simulink model "top_integrated_nanogrid"  (R2026a)
settings: Solver=ode23t  StopTime=1
values from neighbouring files (symbols this model uses):
  irradiance_day = pchip(t_coarse, irradiance_coarse, t_sim)    [flc_init.m]
  t_sim = linspace(0, 1.0, 1001)    [flc_init.m]
undefined symbols (not defined in the file or in its folder): DiscIntNeverNeededParam
libraries: fl_lib x19, nesl_utility x14, ee_lib x13, slpidlib x2, batteryecm_lib x1, fuzblock x1, eePwmGenerator x1
(part 2 of 2)

== matlab function top_integrated_nanogrid/MPPT/MATLAB Function ==
  data: u input; y output
function y = scale_signal(u)
    % Scale [-60, 100] to [-1, 1] with input clamping
    u_clamped = min(max(u, -60), 100); 
    y = (u_clamped - 20) / 80;
end

== matlab function top_integrated_nanogrid/MANAGEMENT_SYSTEM/MATLAB Function ==
  data: P_solar input; Mode output; P_load input; SoC input; P_net output; Battery_Cmd output; Load_Status output
function [Mode, P_net, Battery_Cmd, Load_Status] = nanogrid_controller(P_solar, P_load, SoC)
% #codegen

% --- 1. DEFAULT INITIALIZATIONS (Prevents Undefined Output Errors) ---
Mode        = 1;     % Default to Mode 1
P_net       = 0;     % Default power balance
Battery_Cmd = 0;     % Default Battery Idle (0)
Load_Status = 1;     % Default Load Connected (1)

% --- 2. POWER CALCULATION ---
P_net = P_solar - P_load;

% --- 3. ENERGY MANAGEMENT LOGIC ---
if P_solar >= P_load
    % --- PV Generation Covers or Exceeds Demand ---
    if P_solar == P_load
        % MODE 1: Solar matches load demand perfectly
        Mode = 1;
        Battery_Cmd = 0; % Idle
        
    elseif P_net > 0 && P_load > 0
        % MODE 2: Surplus solar power feeds load and charges battery
        Mode = 2;
        if SoC < 85
            Battery_Cmd = 1; % Charge
        else
            Battery_Cmd = 0; % Battery full, stop charging
        end
        
    else
        % MODE 3: No load connected, full solar power charges battery
        Mode = 3;
        Battery_Cmd = 1; % Charge
    end

else
    % --- Deficit Generation Condition (P_solar < P_load) ---
    if P_solar > 0
        % MODE 4: Partial solar available; Battery supplements load demand
        Mode = 4;
        if SoC > 20
            Battery_Cmd = -1; % Discharge battery
            Load_Status = 1;  % Keep load connected
        else
            Battery_Cmd = 0;  % Stop discharging
            Load_Status = 0;  % Shed load (SoC critically low)
        end

    else
        % MODE 5: Zero solar power; Battery feeds entire load demand
        Mode = 5;
        if SoC > 20
            Battery_Cmd = -1; % Discharge battery
            Load_Status = 1;  % Keep load connected
        else
            Battery_Cmd = 0;  % Stop discharging
            Load_Status = 0;  % Shed load (SoC critically low)
        end
    end
end
